simulink model "F1_Simulator"  (R2026a)
settings: Solver=VariableStepAuto  StopTime=260  MaxStep=0.01
values from neighbouring files (symbols this model uses):
  C = [C; C(1,:)]    [f1_corner_map.m]    (also in f1_lateral_tire_table.m = 1.3; f1_sector_map.m = C([true; hypot(diff(C(:,1)), diff(C(:,2))) > 1e-6], :); f1_sensitivity_sweep.m = {; f1_telemetry.m = C([true; hypot(diff(C(:,1)), diff(C(:,2))) > 1e-6], :))
  m = sU >= d0 & sU <= d1    [f1_corner_map.m]    (also in f1_sector_map.m = dC >= edM(k) & dC <= edM(k+1); f1_speed_profile.m = veh.m)
  normalX = -tangentY    [f1_finish_line_params.m]
  normalY = tangentX    [f1_finish_line_params.m]
  s = cumtrapz(tg, v)    [f1_internal_states.m]    (also in f1_track_animation.m = [0; cumsum(hypot(diff(x), diff(y)))]; f1_track_curvature.m = s_all(keepIdx))
  startX = track(1,1)    [f1_finish_line_params.m]
  startY = track(1,2)    [f1_finish_line_params.m]
  tangentX = dirVec(1)    [f1_finish_line_params.m]
  tangentY = dirVec(2)    [f1_finish_line_params.m]
  trackPsi = psi(idx)    [f1_load_raceline.m]    (also in f1_track_curvature.m = atan2(gradient(trackY), gradient(trackX)))
  trackVref = min(trackVref, vf)    [f1_speed_profile.m]
  trackX = x0    [f1_load_raceline.m]    (also in f1_track_curvature.m = x; silverstone_curvature.mat = [-563.032417564 -561.782952087 -560.539483404 -559.300900612)
  trackY = y0    [f1_load_raceline.m]    (also in f1_track_curvature.m = y; silverstone_curvature.mat = [-515.713759288 -514.151171661 -512.584488731 -511.014091481)
undefined symbols (not defined in the file or in its folder): fp_brk_bore, fp_brk_front, fp_brk_maxT, fp_brk_mu_k, fp_brk_pads, fp_brk_Rm, fp_CdA_corner, fp_CdA_straight, fp_eta_tr, fp_gears, fp_h_cg, fp_mu_brake, fp_mu_pk, fp_mu_trac, fp_N_diff, fp_rho, fp_rpm_dn, fp_rpm_lim_end, fp_rpm_lim_ini, fp_rpm_up, fp_track, pwr, veh
libraries: vehdynlibtire x4, autolibsharedcoupling x3, simulink x1, vehdynlibdriver x1, autolibsharedtransfixedgear x1, autolibshareddiff x1, autolibsharedmappedengines x1, autolibshared x1
(part 1 of 5)
Description:
  | Closed-loop lap simulation of a 2026-regulation Formula 1 car on the Silverstone circuit. A Predictive Driver (Stanley steering + speed-profile tracking) commands a 3-DOF dual-track vehicle with mapped lateral tire tables, a Magic Formula longitudinal tire, an 8-speed gearbox and active aerodynamics (straight mode). A lap timer detects finish-line crossings.
  | 
  | Simulated lap: 94.91 s vs. 88.09 s real (+7.7 %); validated against public telemetry. Built from public data only (regulations, public telemetry, literature).
  | 
  | Initialization: run f1_vehicle_params before simulating.
  | Known limits (rigid body, no ERS, dry track only, lumped aerodynamics) are documented in README_F1_Simulator.md.
  | 
  | Author: Julian Orozco
  | Repository Link: https://github.com/Julian9911
settings Model: Creator=Julian  LastModifiedBy=Julian

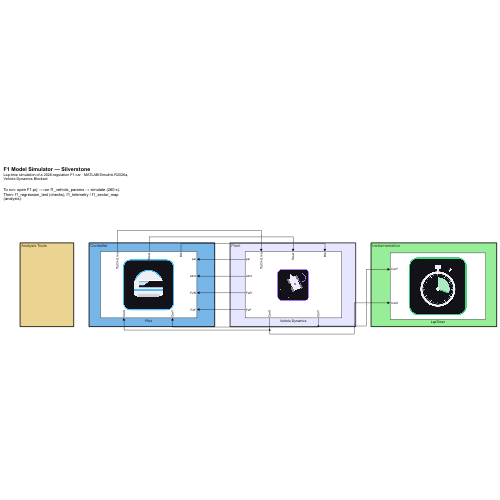
[thumbnail: Simulink's stored preview of the top-level diagram]
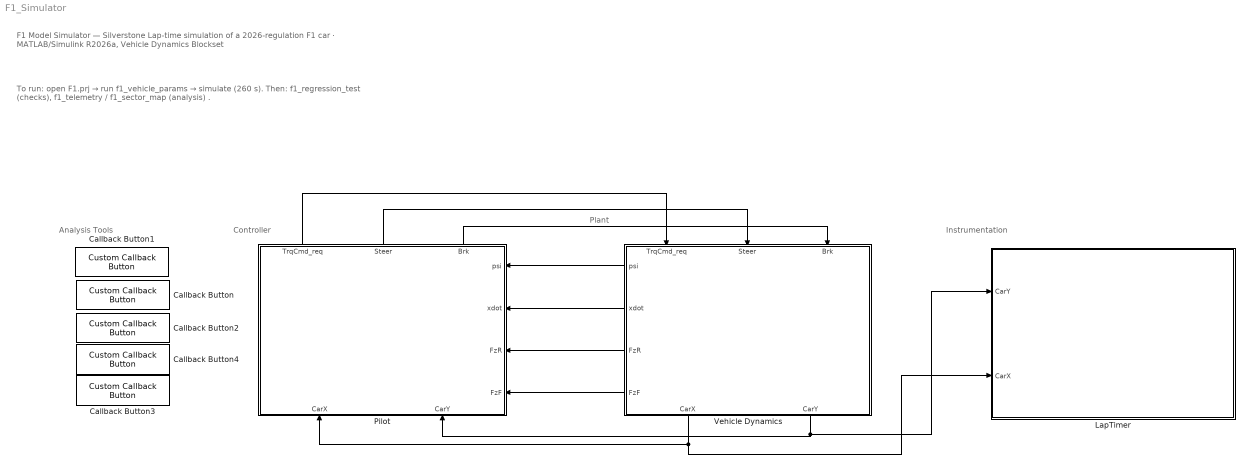
== system F1_Simulator ==
  note: Controller
  note: To run: open F1.prj → run f1_vehicle_params → simulate (260 s).
      | Then: f1_regression_test (checks), f1_telemetry / f1_sector_map (analysis) .
  note: F1 Model Simulator — Silverstone
      | Lap-time simulation of a 2026-regulation F1 car · MATLAB/Simulink R2026a, Vehicle Dynamics Blockset
  note: Plant
  note: Instrumentation
  note: Analysis Tools
  Callback Button : CustomCallbackButton  Configuration="{\"components\":[{\"name\":\"BackgroundImageComponent\",\"settings\":{\"image\":{\"size\":[0,0],\"src\":\"default\",\"srcOrientation\":\"Right\"},\"position\":[0,0,1,1]}},{\"name\":\"ButtonStateComponent\",\"settings\":{\"buttonType\":\"momentary\",\"clickFcn\":\"if ~evalin('base','exist(''out'',''var'')')\\n    warndlg('Run the simulation first.', 'F1 Simulator');\\nelse\\n    evalin('base','f1_telemetry')      % o f1_sector_map \\/ f1_track_animation\\nend\",\"onValue\":1,\"position\":[0,0,1,1],\"pressDelay\":\"500\",\"pressFcn\":\"\",\"repeatInterval\":\"0\",\"states\":[{\"horizontalAlignment\":\"center\",\"image\":{\"position\":[0,0,1,1],\"size\":[1,1],\"src\":\"default\",\"srcOrientation\":\"Right\"},\"label\":{\"color\":[0.01176470588,0.01176470588,0.01176470588,1],\"icon\":{\"size\":[0,0],\"src\":\"default\",\"srcOrientation\":\"Right\"},\"iconOffset\":0,\"iconPlacement\":\"left\",\"opacity\":1,\"show\":true,\"text\":{\"content\":\"Telemetry\",\"font\":\"Helvetica\"}},\"labelOffset\":[0,0],\"verticalAlignment\":\"middle\"},{\"horizontalAlignment\":\"center\",\"image\":{\"position\":[0,0,1,1],\"size\":[1,1],\"src\":\"default\",\"srcOrientation\":\"Right\"},\"label\":{\"color\":[0.01176470588,0.01176470588,0.01176470588,1],\"icon\":{\"size\":[0,0],\"src\":\"default\",\"srcOrientation\":\"Right\"},\"iconOffset\":0,\"iconPlacement\":\"left\",\"opacity\":1,\"show\":true,\"text\":{\"content\":\"Telemetry\",\"font\":\"Helvetica\"}},\"labelOffset\":[0,0],\"verticalAlignment\":\"middle\"},{\"horizontalAlignment\":\"center\",\"image\":{\"position\":[0,0,1,1],\"size\":[1,1],\"src\":\"default\",\"srcOrientation\":\"Right\"},\"label\":{\"color\":[0.01176470588,0.01176470588,0.01176470588,1],\"icon\":{\"size\":[0,0],\"src\":\"default\",\"srcOrientation\":\"Right\"},\"iconOffset\":0,\"iconPlacement\":\"left\",\"opacity\":1,\"show\":true,\"text\":{\"content\":\"Telemetry\",\"font\":\"Helvetica\"}},\"labelOffset\":[0,0],\"verticalAlignment\":\"middle\"},{\"horizontalAlignment\":\"center\",\"image\":{\"position\":[0,0,1,1],\"size\":[1,1],\"src\":\"default\",\"srcOrientation\":\"Right\"},\"label\":{\"color\":[0.01176470588,0.01176470588,0.01176470588,1],\"icon\":{\"size\":[0,0],\"src\":\"default\",\"srcOrientation\":\"Right\"},\"iconOffset\":0,\"iconPlacement\":\"left\",\"opacity\":1,\"show\":true,\"text\":{\"content\":\"Telemetry\",\"font\":\"Helvetica\"}},\"labelOffset\":[0,0],\"verticalAlignment\":\"middle\"}]}},{\"name\":\"ForegroundImageComponent\",\"settings\":{\"image\":{\"size\":[0,0],\"src\":\"default\",\"srcOrientation\":\"Right\"},\"isForeground\":1,\"position\":[0,0,1,1]}}],\"derived\":{\"blockParameters\":{\"AutoActivate\":true,\"ButtonText\":\"Telemetry\",\"ButtonType\":\"Momentary\",\"ClickFcn\":\"if ~evalin('base','exist(''out'',''var'')')\\n    warndlg('Run the simulation first.', 'F1 Simulator');\\nelse\\n    evalin('base','f1_telemetry')      % o f1_sector_map \\/ f1_track_animation\\nend\",\"OnValue\":1,\"PressDelay\":\"500\",\"PressFcn\":\"\",\"RepeatInterval\":\"0\",\"fixedAspectRatio\":\"off\"}},\"settings\":{\"BindingType\":\"standalone\",\"autoActivate\":true,\"backgroundColor\":[244,244,244,1],\"backgroundOffset\":0.2,\"backgroundOpacity\":1,\"fixedAspectRatio\":\"off\",\"foregroundColor\":[0.01176470588,0.01176470588,0.01176470588,1],\"migratedFromLegacy\":true,\"useBackgroundColor\":true,\"variant\":\"callback\",\"version\":\"R2025a\"},\"type\":\"Button\"}"  CustomBackgroundColor="{\"color\":[0.9568627451,0.9568627451,0.9568627451],\"show\":true}"
  Callback Button1 : CustomCallbackButton  Configuration="{\"components\":[{\"name\":\"BackgroundImageComponent\",\"settings\":{\"image\":{\"size\":[0,0],\"src\":\"default\",\"srcOrientation\":\"Right\"},\"position\":[0,0,1,1]}},{\"name\":\"ButtonStateComponent\",\"settings\":{\"buttonType\":\"momentary\",\"clickFcn\":\"if ~evalin('base','exist(''out'',''var'')')\\n    warndlg('Run the simulation first.', 'F1 Simulator');\\nelse\\n    evalin('base','f1_track_animation')      % o f1_sector_map \\/ f1_track_animation\\nend\",\"onValue\":1,\"position\":[0,0,1,1],\"pressDelay\":\"500\",\"pressFcn\":\"\",\"repeatInterval\":\"0\",\"states\":[{\"horizontalAlignment\":\"center\",\"image\":{\"position\":[0,0,1,1],\"size\":[1,1],\"src\":\"default\",\"srcOrientation\":\"Right\"},\"label\":{\"color\":[0.01176470588,0.01176470588,0.01176470588,1],\"icon\":{\"size\":[0,0],\"src\":\"default\",\"srcOrientation\":\"Right\"},\"iconOffset\":0,\"iconPlacement\":\"left\",\"opacity\":1,\"show\":true,\"text\":{\"content\":\"Animation\",\"font\":\"Helvetica\"}},\"labelOffset\":[0,0],\"verticalAlignment\":\"middle\"},{\"horizontalAlignment\":\"center\",\"image\":{\"position\":[0,0,1,1],\"size\":[1,1],\"src\":\"default\",\"srcOrientation\":\"Right\"},\"label\":{\"color\":[0.01176470588,0.01176470588,0.01176470588,1],\"icon\":{\"size\":[0,0],\"src\":\"default\",\"srcOrientation\":\"Right\"},\"iconOffset\":0,\"iconPlacement\":\"left\",\"opacity\":1,\"show\":true,\"text\":{\"content\":\"Animation\",\"font\":\"Helvetica\"}},\"labelOffset\":[0,0],\"verticalAlignment\":\"middle\"},{\"horizontalAlignment\":\"center\",\"image\":{\"position\":[0,0,1,1],\"size\":[1,1],\"src\":\"default\",\"srcOrientation\":\"Right\"},\"label\":{\"color\":[0.01176470588,0.01176470588,0.01176470588,1],\"icon\":{\"size\":[0,0],\"src\":\"default\",\"srcOrientation\":\"Right\"},\"iconOffset\":0,\"iconPlacement\":\"left\",\"opacity\":1,\"show\":true,\"text\":{\"content\":\"Animation\",\"font\":\"Helvetica\"}},\"labelOffset\":[0,0],\"verticalAlignment\":\"middle\"},{\"horizontalAlignment\":\"center\",\"image\":{\"position\":[0,0,1,1],\"size\":[1,1],\"src\":\"default\",\"srcOrientation\":\"Right\"},\"label\":{\"color\":[0.01176470588,0.01176470588,0.01176470588,1],\"icon\":{\"size\":[0,0],\"src\":\"default\",\"srcOrientation\":\"Right\"},\"iconOffset\":0,\"iconPlacement\":\"left\",\"opacity\":1,\"show\":true,\"text\":{\"content\":\"Animation\",\"font\":\"Helvetica\"}},\"labelOffset\":[0,0],\"verticalAlignment\":\"middle\"}]}},{\"name\":\"ForegroundImageComponent\",\"settings\":{\"image\":{\"size\":[0,0],\"src\":\"default\",\"srcOrientation\":\"Right\"},\"isForeground\":1,\"position\":[0,0,1,1]}}],\"derived\":{\"blockParameters\":{\"AutoActivate\":true,\"ButtonText\":\"Animation\",\"ButtonType\":\"Momentary\",\"ClickFcn\":\"if ~evalin('base','exist(''out'',''var'')')\\n    warndlg('Run the simulation first.', 'F1 Simulator');\\nelse\\n    evalin('base','f1_track_animation')      % o f1_sector_map \\/ f1_track_animation\\nend\",\"OnValue\":1,\"PressDelay\":\"500\",\"PressFcn\":\"\",\"RepeatInterval\":\"0\",\"fixedAspectRatio\":\"off\"}},\"settings\":{\"BindingType\":\"standalone\",\"autoActivate\":true,\"backgroundColor\":[244,244,244,1],\"backgroundOffset\":0.2,\"backgroundOpacity\":1,\"fixedAspectRatio\":\"off\",\"foregroundColor\":[0.01176470588,0.01176470588,0.01176470588,1],\"migratedFromLegacy\":true,\"useBackgroundColor\":true,\"variant\":\"callback\",\"version\":\"R2025a\"},\"type\":\"Button\"}"  CustomBackgroundColor="{\"color\":[0.9568627451,0.9568627451,0.9568627451],\"show\":true}"
  Callback Button2 : CustomCallbackButton  Configuration="{\"components\":[{\"name\":\"BackgroundImageComponent\",\"settings\":{\"image\":{\"size\":[0,0],\"src\":\"default\",\"srcOrientation\":\"Right\"},\"position\":[0,0,1,1]}},{\"name\":\"ButtonStateComponent\",\"settings\":{\"buttonType\":\"momentary\",\"clickFcn\":\"if ~evalin('base','exist(''out'',''var'')')\\n    warndlg('Run the simulation first.', 'F1 Simulator');\\nelse\\n    evalin('base','f1_sector_map')      % o f1_sector_map \\/ f1_track_animation\\nend\",\"onValue\":1,\"position\":[0,0,1,1],\"pressDelay\":\"500\",\"pressFcn\":\"\",\"repeatInterval\":\"0\",\"states\":[{\"horizontalAlignment\":\"center\",\"image\":{\"position\":[0,0,1,1],\"size\":[1,1],\"src\":\"default\",\"srcOrientation\":\"Right\"},\"label\":{\"color\":[0.01176470588,0.01176470588,0.01176470588,1],\"icon\":{\"size\":[0,0],\"src\":\"default\",\"srcOrientation\":\"Right\"},\"iconOffset\":0,\"iconPlacement\":\"left\",\"opacity\":1,\"show\":true,\"text\":{\"content\":\"Sector Map\",\"font\":\"Helvetica\"}},\"labelOffset\":[0,0],\"verticalAlignment\":\"middle\"},{\"horizontalAlignment\":\"center\",\"image\":{\"position\":[0,0,1,1],\"size\":[1,1],\"src\":\"default\",\"srcOrientation\":\"Right\"},\"label\":{\"color\":[0.01176470588,0.01176470588,0.01176470588,1],\"icon\":{\"size\":[0,0],\"src\":\"default\",\"srcOrientation\":\"Right\"},\"iconOffset\":0,\"iconPlacement\":\"left\",\"opacity\":1,\"show\":true,\"text\":{\"content\":\"Sector Map\",\"font\":\"Helvetica\"}},\"labelOffset\":[0,0],\"verticalAlignment\":\"middle\"},{\"horizontalAlignment\":\"center\",\"image\":{\"position\":[0,0,1,1],\"size\":[1,1],\"src\":\"default\",\"srcOrientation\":\"Right\"},\"label\":{\"color\":[0.01176470588,0.01176470588,0.01176470588,1],\"icon\":{\"size\":[0,0],\"src\":\"default\",\"srcOrientation\":\"Right\"},\"iconOffset\":0,\"iconPlacement\":\"left\",\"opacity\":1,\"show\":true,\"text\":{\"content\":\"Sector Map\",\"font\":\"Helvetica\"}},\"labelOffset\":[0,0],\"verticalAlignment\":\"middle\"},{\"horizontalAlignment\":\"center\",\"image\":{\"position\":[0,0,1,1],\"size\":[1,1],\"src\":\"default\",\"srcOrientation\":\"Right\"},\"label\":{\"color\":[0.01176470588,0.01176470588,0.01176470588,1],\"icon\":{\"size\":[0,0],\"src\":\"default\",\"srcOrientation\":\"Right\"},\"iconOffset\":0,\"iconPlacement\":\"left\",\"opacity\":1,\"show\":true,\"text\":{\"content\":\"Sector Map\",\"font\":\"Helvetica\"}},\"labelOffset\":[0,0],\"verticalAlignment\":\"middle\"}]}},{\"name\":\"ForegroundImageComponent\",\"settings\":{\"image\":{\"size\":[0,0],\"src\":\"default\",\"srcOrientation\":\"Right\"},\"isForeground\":1,\"position\":[0,0,1,1]}}],\"derived\":{\"blockParameters\":{\"AutoActivate\":true,\"ButtonText\":\"Sector Map\",\"ButtonType\":\"Momentary\",\"ClickFcn\":\"if ~evalin('base','exist(''out'',''var'')')\\n    warndlg('Run the simulation first.', 'F1 Simulator');\\nelse\\n    evalin('base','f1_sector_map')      % o f1_sector_map \\/ f1_track_animation\\nend\",\"OnValue\":1,\"PressDelay\":\"500\",\"PressFcn\":\"\",\"RepeatInterval\":\"0\",\"fixedAspectRatio\":\"off\"}},\"settings\":{\"BindingType\":\"standalone\",\"autoActivate\":true,\"backgroundColor\":[244,244,244,1],\"backgroundOffset\":0.2,\"backgroundOpacity\":1,\"fixedAspectRatio\":\"off\",\"foregroundColor\":[0.01176470588,0.01176470588,0.01176470588,1],\"migratedFromLegacy\":true,\"useBackgroundColor\":true,\"variant\":\"callback\",\"version\":\"R2025a\"},\"type\":\"Button\"}"  CustomBackgroundColor="{\"color\":[0.9568627451,0.9568627451,0.9568627451],\"show\":true}"
  Callback Button3 : CustomCallbackButton  Configuration="{\"components\":[{\"name\":\"BackgroundImageComponent\",\"settings\":{\"image\":{\"size\":[0,0],\"src\":\"default\",\"srcOrientation\":\"Right\"},\"position\":[0,0,1,1]}},{\"name\":\"ButtonStateComponent\",\"settings\":{\"buttonType\":\"momentary\",\"clickFcn\":\"if ~evalin('base','exist(''out'',''var'')')\\n    warndlg('Run the simulation first.', 'F1 Simulator');\\nelse\\n    evalin('base','f1_internal_states')      % o f1_sector_map \\/ f1_track_animation\\nend\",\"onValue\":1,\"position\":[0,0,1,1],\"pressDelay\":\"500\",\"pressFcn\":\"\",\"repeatInterval\":\"0\",\"states\":[{\"horizontalAlignment\":\"center\",\"image\":{\"position\":[0,0,1,1],\"size\":[1,1],\"src\":\"default\",\"srcOrientation\":\"Right\"},\"label\":{\"color\":[0.01176470588,0.01176470588,0.01176470588,1],\"icon\":{\"size\":[0,0],\"src\":\"default\",\"srcOrientation\":\"Right\"},\"iconOffset\":0,\"iconPlacement\":\"left\",\"opacity\":1,\"show\":true,\"text\":{\"content\":\"Internal States\",\"font\":\"Helvetica\"}},\"labelOffset\":[0,0],\"verticalAlignment\":\"middle\"},{\"horizontalAlignment\":\"center\",\"image\":{\"position\":[0,0,1,1],\"size\":[1,1],\"src\":\"default\",\"srcOrientation\":\"Right\"},\"label\":{\"color\":[0.01176470588,0.01176470588,0.01176470588,1],\"icon\":{\"size\":[0,0],\"src\":\"default\",\"srcOrientation\":\"Right\"},\"iconOffset\":0,\"iconPlacement\":\"left\",\"opacity\":1,\"show\":true,\"text\":{\"content\":\"Internal States\",\"font\":\"Helvetica\"}},\"labelOffset\":[0,0],\"verticalAlignment\":\"middle\"},{\"horizontalAlignment\":\"center\",\"image\":{\"position\":[0,0,1,1],\"size\":[1,1],\"src\":\"default\",\"srcOrientation\":\"Right\"},\"label\":{\"color\":[0.01176470588,0.01176470588,0.01176470588,1],\"icon\":{\"size\":[0,0],\"src\":\"default\",\"srcOrientation\":\"Right\"},\"iconOffset\":0,\"iconPlacement\":\"left\",\"opacity\":1,\"show\":true,\"text\":{\"content\":\"Internal States\",\"font\":\"Helvetica\"}},\"labelOffset\":[0,0],\"verticalAlignment\":\"middle\"},{\"horizontalAlignment\":\"center\",\"image\":{\"position\":[0,0,1,1],\"size\":[1,1],\"src\":\"default\",\"srcOrientation\":\"Right\"},\"label\":{\"color\":[0.01176470588,0.01176470588,0.01176470588,1],\"icon\":{\"size\":[0,0],\"src\":\"default\",\"srcOrientation\":\"Right\"},\"iconOffset\":0,\"iconPlacement\":\"left\",\"opacity\":1,\"show\":true,\"text\":{\"content\":\"Internal States\",\"font\":\"Helvetica\"}},\"labelOffset\":[0,0],\"verticalAlignment\":\"middle\"}]}},{\"name\":\"ForegroundImageComponent\",\"settings\":{\"image\":{\"size\":[0,0],\"src\":\"default\",\"srcOrientation\":\"Right\"},\"isForeground\":1,\"position\":[0,0,1,1]}}],\"derived\":{\"blockParameters\":{\"AutoActivate\":true,\"ButtonText\":\"Internal States\",\"ButtonType\":\"Momentary\",\"ClickFcn\":\"if ~evalin('base','exist(''out'',''var'')')\\n    warndlg('Run the simulation first.', 'F1 Simulator');\\nelse\\n    evalin('base','f1_internal_states')      % o f1_sector_map \\/ f1_track_animation\\nend\",\"OnValue\":1,\"PressDelay\":\"500\",\"PressFcn\":\"\",\"RepeatInterval\":\"0\",\"fixedAspectRatio\":\"off\"}},\"settings\":{\"BindingType\":\"standalone\",\"autoActivate\":true,\"backgroundColor\":[244,244,244,1],\"backgroundOffset\":0.2,\"backgroundOpacity\":1,\"fixedAspectRatio\":\"off\",\"foregroundColor\":[0.01176470588,0.01176470588,0.01176470588,1],\"migratedFromLegacy\":true,\"useBackgroundColor\":true,\"variant\":\"callback\",\"version\":\"R2025a\"},\"type\":\"Button\"}"  CustomBackgroundColor="{\"color\":[0.9568627451,0.9568627451,0.9568627451],\"show\":true}"
  Callback Button4 : CustomCallbackButton  Configuration="{\"components\":[{\"name\":\"BackgroundImageComponent\",\"settings\":{\"image\":{\"size\":[0,0],\"src\":\"default\",\"srcOrientation\":\"Right\"},\"position\":[0,0,1,1]}},{\"name\":\"ButtonStateComponent\",\"settings\":{\"buttonType\":\"momentary\",\"clickFcn\":\"if ~evalin('base','exist(''out'',''var'')')\\n    warndlg('Run the simulation first.', 'F1 Simulator');\\nelse\\n    evalin('base','f1_corner_map')      % o f1_sector_map \\/ f1_track_animation\\nend\",\"onValue\":1,\"position\":[0,0,1,1],\"pressDelay\":\"500\",\"pressFcn\":\"\",\"repeatInterval\":\"0\",\"states\":[{\"horizontalAlignment\":\"center\",\"image\":{\"position\":[0,0,1,1],\"size\":[1,1],\"src\":\"default\",\"srcOrientation\":\"Right\"},\"label\":{\"color\":[0.01176470588,0.01176470588,0.01176470588,1],\"icon\":{\"size\":[0,0],\"src\":\"default\",\"srcOrientation\":\"Right\"},\"iconOffset\":0,\"iconPlacement\":\"left\",\"opacity\":1,\"show\":true,\"text\":{\"content\":\"Corner Map\",\"font\":\"Helvetica\"}},\"labelOffset\":[0,0],\"verticalAlignment\":\"middle\"},{\"horizontalAlignment\":\"center\",\"image\":{\"position\":[0,0,1,1],\"size\":[1,1],\"src\":\"default\",\"srcOrientation\":\"Right\"},\"label\":{\"color\":[0.01176470588,0.01176470588,0.01176470588,1],\"icon\":{\"size\":[0,0],\"src\":\"default\",\"srcOrientation\":\"Right\"},\"iconOffset\":0,\"iconPlacement\":\"left\",\"opacity\":1,\"show\":true,\"text\":{\"content\":\"Corner Map\",\"font\":\"Helvetica\"}},\"labelOffset\":[0,0],\"verticalAlignment\":\"middle\"},{\"horizontalAlignment\":\"center\",\"image\":{\"position\":[0,0,1,1],\"size\":[1,1],\"src\":\"default\",\"srcOrientation\":\"Right\"},\"label\":{\"color\":[0.01176470588,0.01176470588,0.01176470588,1],\"icon\":{\"size\":[0,0],\"src\":\"default\",\"srcOrientation\":\"Right\"},\"iconOffset\":0,\"iconPlacement\":\"left\",\"opacity\":1,\"show\":true,\"text\":{\"content\":\"Corner Map\",\"font\":\"Helvetica\"}},\"labelOffset\":[0,0],\"verticalAlignment\":\"middle\"},{\"horizontalAlignment\":\"center\",\"image\":{\"position\":[0,0,1,1],\"size\":[1,1],\"src\":\"default\",\"srcOrientation\":\"Right\"},\"label\":{\"color\":[0.01176470588,0.01176470588,0.01176470588,1],\"icon\":{\"size\":[0,0],\"src\":\"default\",\"srcOrientation\":\"Right\"},\"iconOffset\":0,\"iconPlacement\":\"left\",\"opacity\":1,\"show\":true,\"text\":{\"content\":\"Corner Map\",\"font\":\"Helvetica\"}},\"labelOffset\":[0,0],\"verticalAlignment\":\"middle\"}]}},{\"name\":\"ForegroundImageComponent\",\"settings\":{\"image\":{\"size\":[0,0],\"src\":\"default\",\"srcOrientation\":\"Right\"},\"isForeground\":1,\"position\":[0,0,1,1]}}],\"derived\":{\"blockParameters\":{\"AutoActivate\":true,\"ButtonText\":\"Corner Map\",\"ButtonType\":\"Momentary\",\"ClickFcn\":\"if ~evalin('base','exist(''out'',''var'')')\\n    warndlg('Run the simulation first.', 'F1 Simulator');\\nelse\\n    evalin('base','f1_corner_map')      % o f1_sector_map \\/ f1_track_animation\\nend\",\"OnValue\":1,\"PressDelay\":\"500\",\"PressFcn\":\"\",\"RepeatInterval\":\"0\",\"fixedAspectRatio\":\"off\"}},\"settings\":{\"BindingType\":\"standalone\",\"autoActivate\":true,\"backgroundColor\":[244,244,244,1],\"backgroundOffset\":0.2,\"backgroundOpacity\":1,\"fixedAspectRatio\":\"off\",\"foregroundColor\":[0.01176470588,0.01176470588,0.01176470588,1],\"migratedFromLegacy\":true,\"useBackgroundColor\":true,\"variant\":\"callback\",\"version\":\"R2025a\"},\"type\":\"Button\"}"  CustomBackgroundColor="{\"color\":[0.9568627451,0.9568627451,0.9568627451],\"show\":true}"
  LapTimer : Subsystem
      mask Display: image('icon_crono.png', [0,0,0,0,90,90]);
  Pilot : Subsystem
      settings: PortSchema="{\"entries\":[{\"content\":{\"sides\":[{\"content\":{},\"type\":\"ConnectorPlacement.EquallySpacedRectSide\",\"uuid\":\"6dbb380a-1e16-4c70-a0b7-134b981a2922\"},{\"content\":{\"connectorIds\":[\"In3\",\"In4\",\"In5\",\"In6\"],\"side\":\"RIGHT\"},\"type\":\"ConnectorPlacement.EquallySpacedRectSide\",\"uuid\":\"1d819d40-d3d8-4f1d-853d-b565b7154945\"},{\"content\":{\"connectorIds\":[\"Out1\",\"Out2\",\"Out3\"],\"side\":\"TOP\"},\"type\":\"ConnectorPlacement.EquallySpacedRectSide\",\"uuid\":\"0a78c45d-d0d8-410b-afc8-98defaac373b\"},{\"content\":{\"connectorIds\":[\"In1\",\"In2\"],\"side\":\"BOTTOM\"},\"type\":\"ConnectorPlacement.EquallySpacedRectSide\",\"uuid\":\"7781406f-9023-43c1-9af0-81ef65fd786b\"}]},\"type\":\"ConnectorPlacement.EquallySpacedConnector\",\"uuid\":\"ad0d07c2-c40c-4492-9b2d-a3520ec4bf64\"}],\"packageUris\":[\"http://schema.mathworks.com/mf0/Connector/R2020b\"],\"version\":\"1.0\"}"
      mask Display: image('icon_pilot.png', [0,0,0,0,80,80]);
  Vehicle Dynamics : Subsystem
      settings: PortSchema="{\"entries\":[{\"content\":{\"sides\":[{\"content\":{\"connectorIds\":[\"Out3\",\"Out4\",\"Out5\",\"Out6\"]},\"type\":\"ConnectorPlacement.EquallySpacedRectSide\",\"uuid\":\"755fdee6-d20b-4cca-9328-90816d5527bd\"},{\"content\":{\"side\":\"RIGHT\"},\"type\":\"ConnectorPlacement.EquallySpacedRectSide\",\"uuid\":\"2468d4ca-4565-46a3-a939-cc2d7b98973a\"},{\"content\":{\"connectorIds\":[\"In1\",\"In2\",\"In3\"],\"side\":\"TOP\"},\"type\":\"ConnectorPlacement.EquallySpacedRectSide\",\"uuid\":\"a01d3726-5ed7-4570-a8f3-9e61b58ffa15\"},{\"content\":{\"connectorIds\":[\"Out1\",\"Out2\"],\"side\":\"BOTTOM\"},\"type\":\"ConnectorPlacement.EquallySpacedRectSide\",\"uuid\":\"f3ee33bc-6d92-4657-b545-f57da25f2dbd\"}]},\"type\":\"ConnectorPlacement.EquallySpacedConnector\",\"uuid\":\"32c5194d-a553-427a-bae0-317c328303b5\"}],\"packageUris\":[\"http://schema.mathworks.com/mf0/Connector/R2020b\"],\"version\":\"1.0\"}"
      mask Display: image('icon_vehicle_dynamics.png', [0,0,0,0,50,50]);
  wires:
  Vehicle Dynamics/1(CarX) -> Pilot/1(CarX), LapTimer/2(CarX)
  Vehicle Dynamics/2(CarY) -> Pilot/2(CarY), LapTimer/1(CarY)
  Vehicle Dynamics/4(xdot) -> Pilot/4(xdot)
  Vehicle Dynamics/6(FzF) -> Pilot/6(FzF)
  Vehicle Dynamics/5(FzR) -> Pilot/5(FzR)
  Vehicle Dynamics/3(psi) -> Pilot/3(psi)
  Pilot/1(TrqCmd_req) -> Vehicle Dynamics/1(TrqCmd_req)
  Pilot/3(Brk) -> Vehicle Dynamics/3(Brk)
  Pilot/2(Steer) -> Vehicle Dynamics/2(Steer)

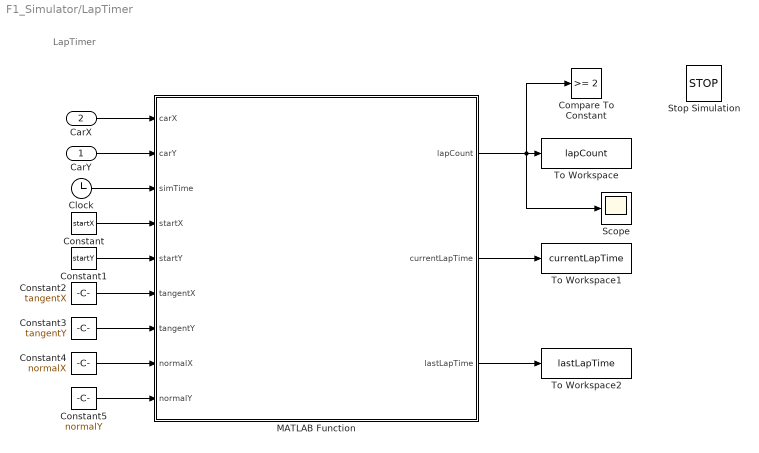
== system F1_Simulator/LapTimer ==
  note: LapTimer
  CarY : Inport
  CarX : Inport  Port=2
  Clock : Clock
  Compare To Constant : simulink/Logic and Bit Operations/Compare To Constant  relop=>=  const=2  OutDataTypeStr=boolean
  Constant : Constant  Value=startX
  Constant1 : Constant  Value=startY
  Constant2 : Constant  Value=tangentX
  Constant3 : Constant  Value=tangentY
  Constant4 : Constant  Value=normalX
  Constant5 : Constant  Value=normalY
  MATLAB Function : MATLAB Function  TreatAsAtomicUnit=on
  Scope : Scope
      settings: ActiveDisplayYMinimum=-1  ActiveDisplayYMaximum=1
  Stop Simulation : Stop
  To Workspace : ToWorkspace  VariableName=lapCount  SaveFormat=Timeseries  SampleTime=-1
  To Workspace1 : ToWorkspace  VariableName=currentLapTime  SaveFormat=Timeseries  SampleTime=-1
  To Workspace2 : ToWorkspace  VariableName=lastLapTime  SaveFormat=Timeseries  SampleTime=-1
  wires:
  MATLAB Function/1(lapCount) -> Scope/1, Compare To Constant/1, To Workspace/1
  MATLAB Function/2(currentLapTime) -> To Workspace1/1
  MATLAB Function/3(lastLapTime) -> To Workspace2/1
  Clock/1 -> MATLAB Function/3(simTime)
  Constant/1 -> MATLAB Function/4(startX)
  Constant1/1 -> MATLAB Function/5(startY)
  Constant2/1 -> MATLAB Function/6(tangentX)
  Constant3/1 -> MATLAB Function/7(tangentY)
  Constant4/1 -> MATLAB Function/8(normalX)
  Constant5/1 -> MATLAB Function/9(normalY)
  CarY/1 -> MATLAB Function/2(carY)
  CarX/1 -> MATLAB Function/1(carX)

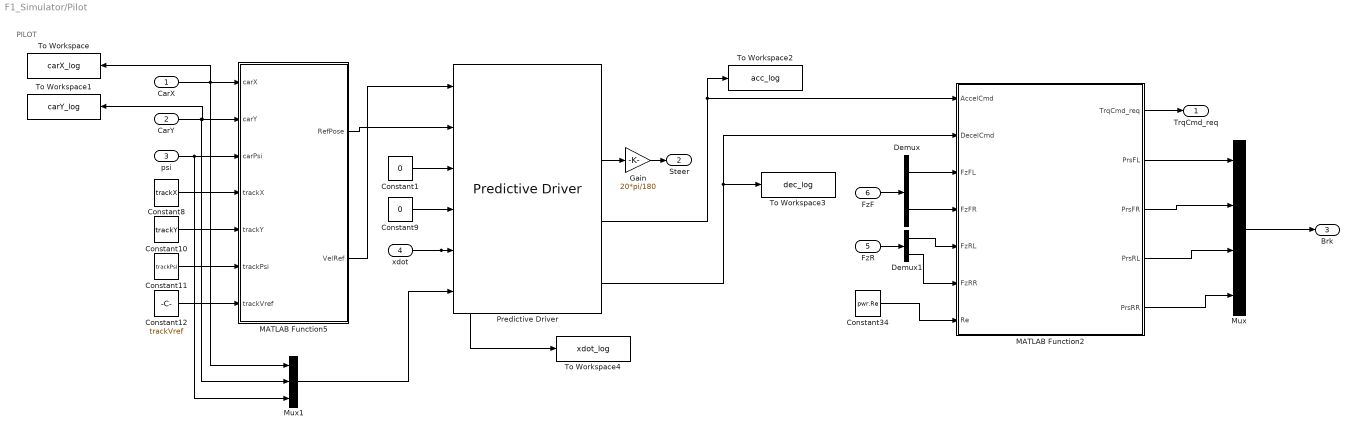
== system F1_Simulator/Pilot ==
  note: PILOT
  CarX : Inport
  CarY : Inport  Port=2
  psi : Inport  Port=3
  xdot : Inport  Port=4
  FzR : Inport  Port=5
  FzF : Inport  Port=6
  Constant1 : Constant  Value=0  OutDataTypeStr=boolean
  Constant10 : Constant  Value=trackY
  Constant11 : Constant  Value=trackPsi
  Constant12 : Constant  Value=trackVref
  Constant34 : Constant  Value=pwr.Re
  Constant8 : Constant  Value=trackX
  Constant9 : Constant  Value=0  OutDataTypeStr=double
  Demux : Demux  Outputs=2
  Demux1 : Demux  Outputs=2
  Gain : Gain  Gain=20*pi/180
  MATLAB Function2 : MATLAB Function  TreatAsAtomicUnit=on
  MATLAB Function5 : MATLAB Function  TreatAsAtomicUnit=on
  Mux : Mux
  Mux1 : Mux  Inputs=3
  Predictive Driver : vehdynlibdriver/Predictive Driver  extAccelOvr=off  extDecelOvr=off  extAccelHld=off  extDecelHld=off  extAccelZero=off  extDecelZero=off  extSteerOvr=off  extSteerHld=off  extSteerZero=on  cntrlType=PI  cntrlTypeLat=Stanley  shftType=None  coordMode=SAE J670 (Z-down)  refType=Reference pose  velUnits=m/s  angUnits=rad  gearOut=off  steerOut=off  Kp=10  Ki=5  Kff=.1  Kg=0  VehVelVec=[0 100]  KffVec=[.1 .1]  KpVec=[10 10]  KiVec=[5 5]  KgVec=[0 0]  vnom=30  Kaw=1  tauerr=0.1  tau=0.1  L=40  Kpt=3000  aR=200  bR=2.5  cR=.5  g=9.81  vecPose=on  dynamMode=off  PositionGainF=2.5  PositionGainR=2.5  YawRateGain=.2  DelayGain=.2  enableDrift=off  BetaRef=20*pi/180  KpBeta=1  KpDrift=2  KdDrift=1  KpPsi=6  KOmega=30  tOmega=1  a=1.87  b=1.53  m=veh.m  Cy_f=50e3  Cy_r=76e3  I=veh.Izz  Ksteer=18  theta=20*pi/180  Idl=3  Re=.3  lambda_mu=1  GearInit=0  tShift=.1  pdlVec=[0.1 0.4 0.5 0.9]  upShftTbl=[-1 12.9375 26.4375 39.9375 51.18749999999999 62.4375 72.84375 83.25;-1 16.3125 29.8125 43.3125 54.5624 65.8125 76.78125 87.75;-1 19.6875 33.1875 46.68749999999999 57.9375 69.1875 80.71875 92.25;-1 33 52.5 77.25 100.5 138.75 161.875 185]  dwnShftTbl=[-1 12.9375 26.4375 39.9375 51.18749999999999 62.4375 72.84375 83.25;-1 16.3125 29.8125 43.3125 54.5624 65.8125 76.78125 87.75;-1 19.6875 33.1875 46.68749999999999 57.9375 69.1875 80.71875 92.25;-1 33 52.5 77.25 100.5 138.75 161.875 185]  tClutch=.5  tRev=.5  tPark=120  UpGearVec="[0  1  2  3  4  5  6  7]"  DownGearVec="[1  2  3  4  5  6  7  8]"  aMode=2
  To Workspace : ToWorkspace  VariableName=carX_log  SaveFormat=Timeseries  SampleTime=-1
  To Workspace1 : ToWorkspace  VariableName=carY_log  SaveFormat=Timeseries  SampleTime=-1
  To Workspace2 : ToWorkspace  VariableName=acc_log  SaveFormat=Timeseries  SampleTime=-1
  To Workspace3 : ToWorkspace  VariableName=dec_log  SaveFormat=Timeseries  SampleTime=-1
  To Workspace4 : ToWorkspace  VariableName=xdot_log  SaveFormat=Timeseries  SampleTime=-1
  TrqCmd_req : Outport
  Steer : Outport  Port=2
  Brk : Outport  Port=3
  wires:
  Constant1/1 -> Predictive Driver/3
  Predictive Driver/3 -> To Workspace2/1, MATLAB Function2/1(AccelCmd)
  Predictive Driver/4 -> To Workspace3/1, MATLAB Function2/2(DecelCmd)
  FzF/1 -> Demux/1
  FzR/1 -> Demux1/1
  Demux/1 -> MATLAB Function2/3(FzFL)
  Demux/2 -> MATLAB Function2/4(FzFR)
  Demux1/1 -> MATLAB Function2/5(FzRL)
  Demux1/2 -> MATLAB Function2/6(FzRR)
  Constant34/1 -> MATLAB Function2/7(Re)
  MATLAB Function2/1(TrqCmd_req) -> TrqCmd_req/1
  MATLAB Function2/2(PrsFL) -> Mux/1
  MATLAB Function2/3(PrsFR) -> Mux/2
  MATLAB Function2/4(PrsRL) -> Mux/3
  MATLAB Function2/5(PrsRR) -> Mux/4
  Constant9/1 -> Predictive Driver/4
  Mux/1 -> Brk/1
  Predictive Driver/2 -> Gain/1
  Gain/1 -> Steer/1
  MATLAB Function5/1(RefPose) -> Predictive Driver/2
  CarY/1 -> To Workspace1/1, MATLAB Function5/2(carY), Mux1/2
  psi/1 -> Mux1/3, MATLAB Function5/3(carPsi)
  Mux1/1 -> Predictive Driver/6
  xdot/1 -> To Workspace4/1, Predictive Driver/5
  Constant8/1 -> MATLAB Function5/4(trackX)
  Constant10/1 -> MATLAB Function5/5(trackY)
  Constant11/1 -> MATLAB Function5/6(trackPsi)
  CarX/1 -> To Workspace/1, Mux1/1, MATLAB Function5/1(carX)
  MATLAB Function5/2(VelRef) -> Predictive Driver/1
  Constant12/1 -> MATLAB Function5/7(trackVref)

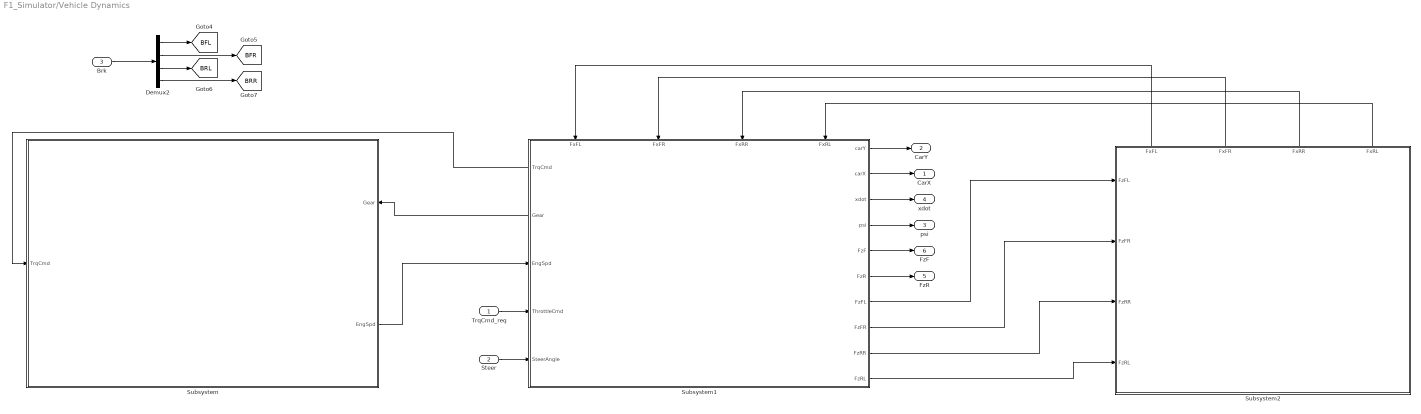
== system F1_Simulator/Vehicle Dynamics ==
  TrqCmd_req : Inport
  Steer : Inport  Port=2
  Brk : Inport  Port=3
  Demux2 : Demux
  Subsystem : Subsystem
      settings: PortSchema="{\"entries\":[{\"content\":{\"sides\":[{\"content\":{\"connectorIds\":[\"In1\"]},\"type\":\"ConnectorPlacement.EquallySpacedRectSide\",\"uuid\":\"382126b2-f943-4b64-b98b-5bd52ec92c72\"},{\"content\":{\"connectorIds\":[\"In2\",\"Out1\"],\"side\":\"RIGHT\"},\"type\":\"ConnectorPlacement.EquallySpacedRectSide\",\"uuid\":\"f48de981-f6df-4a54-bd6d-3aaae0b68c2e\"},{\"content\":{\"side\":\"TOP\"},\"type\":\"ConnectorPlacement.EquallySpacedRectSide\",\"uuid\":\"65130d79-e275-483c-ad87-eca04c403bfa\"}]},\"type\":\"ConnectorPlacement.EquallySpacedConnector\",\"uuid\":\"feba05f0-61cb-4342-bc98-1f604655dd4f\"}],\"packageUris\":[\"http://schema.mathworks.com/mf0/Connector/R2020b\"],\"version\":\"1.0\"}"
      mask Display: image('icon_powertrain.png', [0,0,0,0,70,70]);
  Subsystem1 : Subsystem
      settings: PortSchema="{\"entries\":[{\"content\":{\"sides\":[{\"content\":{\"connectorIds\":[\"Out11\",\"Out12\",\"In1\",\"In2\",\"In3\"]},\"type\":\"ConnectorPlacement.EquallySpacedRectSide\",\"uuid\":\"a8604498-54a6-4e2a-8f7f-86cc2403bbb5\"},{\"content\":{\"connectorIds\":[\"Out1\",\"Out2\",\"Out3\",\"Out4\",\"Out5\",\"Out6\",\"Out7\",\"Out8\",\"Out9\",\"Out10\"],\"side\":\"RIGHT\"},\"type\":\"ConnectorPlacement.EquallySpacedRectSide\",\"uuid\":\"f1a41939-3a8d-4b55-967e-fb3e703e919e\"},{\"content\":{\"connectorIds\":[\"In4\",\"In5\",\"In6\",\"In7\"],\"side\":\"TOP\"},\"type\":\"ConnectorPlacement.EquallySpacedRectSide\",\"uuid\":\"38922609-117e-43d8-a828-713f65c721f6\"}]},\"type\":\"ConnectorPlacement.EquallySpacedConnector\",\"uuid\":\"48326796-8402-4034-b482-1683d1631c02\"}],\"packageUris\":[\"http://schema.mathworks.com/mf0/Connector/R2020b\"],\"version\":\"1.0\"}"
      mask Display: image('icon_vehicle.png', [0,0,0,0,70,70]);
  Subsystem2 : Subsystem
      settings: PortSchema="{\"entries\":[{\"content\":{\"sides\":[{\"content\":{\"connectorIds\":[\"In1\",\"In2\",\"In3\",\"In4\"]},\"type\":\"ConnectorPlacement.EquallySpacedRectSide\",\"uuid\":\"78526832-4c85-4cd7-80b8-0662b4d81380\"},{\"content\":{\"side\":\"RIGHT\"},\"type\":\"ConnectorPlacement.EquallySpacedRectSide\",\"uuid\":\"a734da9d-a3a3-4c82-affb-b775f245601f\"},{\"content\":{\"connectorIds\":[\"Out1\",\"Out2\",\"Out3\",\"Out4\"],\"side\":\"TOP\"},\"type\":\"ConnectorPlacement.EquallySpacedRectSide\",\"uuid\":\"79a0aced-5143-4f3d-9c41-ab235d5ae659\"}]},\"type\":\"ConnectorPlacement.EquallySpacedConnector\",\"uuid\":\"68fca9d3-2a7d-4160-bdc3-3a246dbd5f95\"}],\"packageUris\":[\"http://schema.mathworks.com/mf0/Connector/R2020b\"],\"version\":\"1.0\"}"
      mask Display: image('icon_tires.png', [0,0,0,0,70,70]);
  CarX : Outport
  CarY : Outport  Port=2
  psi : Outport  Port=3
  xdot : Outport  Port=4
  FzR : Outport  Port=5
  FzF : Outport  Port=6
  tag scope: BFL=global, BFR=global, BRL=global, BRR=global
  wires:
  Brk/1 -> Demux2/1
  Demux2/1 -> [BFL]
  Demux2/2 -> [BFR]
  Demux2/3 -> [BRL]
  Demux2/4 -> [BRR]
  Steer/1 -> Subsystem1/3(SteerAngle)
  TrqCmd_req/1 -> Subsystem1/2(ThrottleCmd)
  Subsystem/1(EngSpd) -> Subsystem1/1(EngSpd)
  Subsystem1/1(carY) -> CarY/1
  Subsystem1/2(carX) -> CarX/1
  Subsystem1/3(xdot) -> xdot/1
  Subsystem1/4(psi) -> psi/1
  Subsystem1/5(FzF) -> FzF/1
  Subsystem1/6(FzR) -> FzR/1
  Subsystem1/12(Gear) -> Subsystem/2(Gear)
  Subsystem1/11(TrqCmd) -> Subsystem/1(TrqCmd)
  Subsystem1/7(FzFL) -> Subsystem2/1(FzFL)
  Subsystem1/8(FzFR) -> Subsystem2/2(FzFR)
  Subsystem1/9(FzRR) -> Subsystem2/3(FzRR)
  Subsystem1/10(FzRL) -> Subsystem2/4(FzRL)
  Subsystem2/1(FxFL) -> Subsystem1/4(FxFL)
  Subsystem2/2(FxFR) -> Subsystem1/5(FxFR)
  Subsystem2/3(FxRR) -> Subsystem1/6(FxRR)
  Subsystem2/4(FxRL) -> Subsystem1/7(FxRL)
